simulink model "fw_can1_codec"  (R2026b)
settings: Solver=VariableStepAuto
undefined symbols (not defined in the file or in its folder): P, Ts
libraries: simulink x4
settings Model: Creator=aomar  LastModifiedBy=aomar

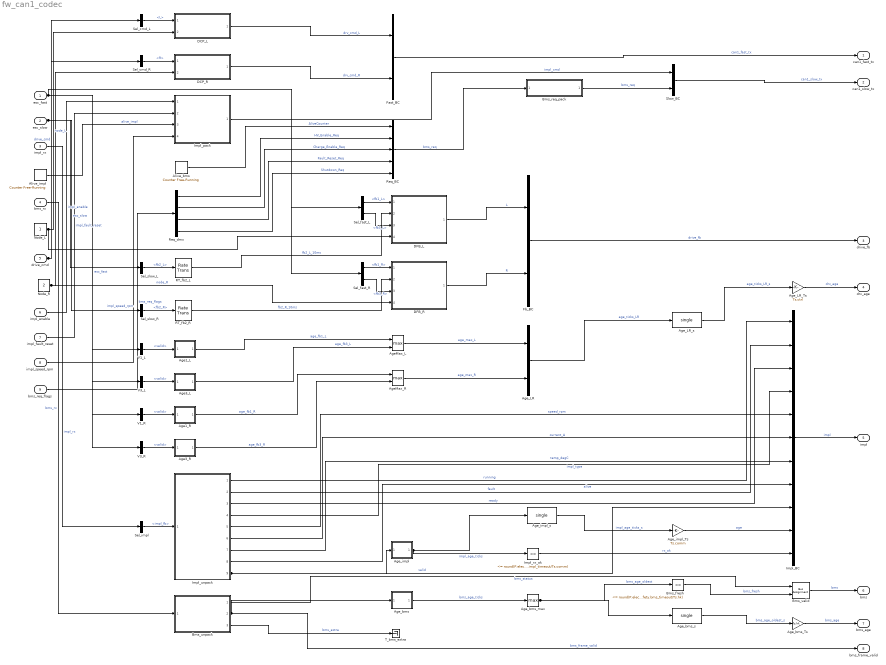
== system fw_can1_codec ==
  esc_fast : Inport  OutDataTypeStr=Bus: Bus_Can1_EscFast  SampleTime=Ts.ctrl
  esc_slow : Inport  Port=2  OutDataTypeStr=Bus: Bus_Can1_EscSlow  SampleTime=Ts.comm
  impl_rx : Inport  Port=3  OutDataTypeStr=Bus: Bus_Can1_Impl  SampleTime=Ts.comm
  bms_rx : Inport  Port=4  OutDataTypeStr=Bus: Bus_Can1_Bms  SampleTime=Ts.hk
  drive_cmd : Inport  Port=5  OutDataTypeStr=Bus: Bus_DriveCmd  SampleTime=Ts.ctrl
  impl_enable : Inport  Port=6  OutDataTypeStr=boolean  SampleTime=Ts.comm
  impl_fault_reset : Inport  Port=7  OutDataTypeStr=boolean  SampleTime=Ts.comm
  impl_speed_rpm : Inport  Port=8  OutDataTypeStr=single  SampleTime=Ts.comm
  bms_req_flags : Inport  Port=9  OutDataTypeStr=boolean  PortDimensions=4  SampleTime=Ts.comm
  Age1_L : Subsystem
  Age1_R : Subsystem
  Age3_L : Subsystem
  Age3_R : Subsystem
  AgeMax_L : MinMax  Function=max  Inputs=2
  AgeMax_R : MinMax  Function=max  Inputs=2
  Age_LR : Concatenate
  Age_LR_Ts : Gain  Gain=Ts.ctrl
  Age_LR_s : DataTypeConversion  OutDataTypeStr=single  RndMeth=Round
  Age_bms : Subsystem
  Age_bms_Ts : Gain  Gain=Ts.hk
  Age_bms_max : MinMax  Function=max
  Age_bms_s : DataTypeConversion  OutDataTypeStr=single  RndMeth=Round
  Age_impl : Subsystem
  Age_impl_Ts : Gain  Gain=Ts.comm
  Age_impl_s : DataTypeConversion  OutDataTypeStr=single  RndMeth=Round
  Alive_bms : simulink/Sources/Counter Free-Running  NumBits=8  tsamp=Ts.comm
  Alive_impl : simulink/Sources/Counter Free-Running  NumBits=8  tsamp=Ts.comm
  Bms_fresh : simulink/Logic and Bit Operations/Compare To Constant  relop=<=  const=round(P.electronics.safety.bms_timeout/Ts.hk)  OutDataTypeStr=boolean
  Bms_req_pack : Subsystem  ReferencedSubsystem=bmsreq_can_pack
  Bms_unpack : Subsystem  ReferencedSubsystem=bms_can_unpack
  Bms_valid : BusAssignment  AssignedSignals=valid
  DCP_L : Subsystem  ReferencedSubsystem=drive_cmd_pack
  DCP_R : Subsystem  ReferencedSubsystem=drive_cmd_pack
  DFB_L : Subsystem  ReferencedSubsystem=drive_fb_unpack
  DFB_R : Subsystem  ReferencedSubsystem=drive_fb_unpack
  Fast_BC : BusCreator  Inputs=2  OutDataTypeStr=Bus: Bus_Can1_McuFast  NonVirtualBus=on
      settings: InheritFromInputs=off
  Fb_BC : BusCreator  Inputs=2  OutDataTypeStr=Bus: Bus_DriveFb  NonVirtualBus=on
      settings: InheritFromInputs=off
  Impl_BC : BusCreator  Inputs=11
  Impl_pack : Subsystem  ReferencedSubsystem=implcmd_can_pack
  Impl_rx_ok : simulink/Logic and Bit Operations/Compare To Constant  relop=<=  const=round(P.electronics.safety.impl_timeout/Ts.comm)  OutDataTypeStr=boolean
  Impl_unpack : Subsystem  ReferencedSubsystem=implfb_can_unpack
  Node_L : Constant  OutDataTypeStr=uint8  SampleTime=-1
  Node_R : Constant  Value=2  OutDataTypeStr=uint8  SampleTime=-1
  RT_fb2_L : RateTransition  InitialCondition=P.ic.Bus_CanFrame8  OutPortSampleTime=Ts.ctrl
  RT_fb2_R : RateTransition  InitialCondition=P.ic.Bus_CanFrame8  OutPortSampleTime=Ts.ctrl
  Req_BC : BusCreator  Inputs=5  OutDataTypeStr=Bus: Bus_BmsReq  NonVirtualBus=on
      settings: InheritFromInputs=off
  Req_dmx : Demux
  Sel_cmd_L : BusSelector  OutputSignals=L
  Sel_cmd_R : BusSelector  OutputSignals=R
  Sel_fast_L : BusSelector  OutputSignals=fb1_L,fb3_L
  Sel_fast_R : BusSelector  OutputSignals=fb1_R,fb3_R
  Sel_impl : BusSelector  OutputSignals=impl_fb
  Sel_slow_L : BusSelector  OutputSignals=fb2_L
  Sel_slow_R : BusSelector  OutputSignals=fb2_R
  Slow_BC : BusCreator  Inputs=2  OutDataTypeStr=Bus: Bus_Can1_McuSlow  NonVirtualBus=on
      settings: InheritFromInputs=off
  T_bms_extra : Terminator
  V1_L : BusSelector  OutputSignals=fb1_L.valid
  V1_R : BusSelector  OutputSignals=fb1_R.valid
  V3_L : BusSelector  OutputSignals=fb3_L.valid
  V3_R : BusSelector  OutputSignals=fb3_R.valid
  can1_fast_tx : Outport  OutDataTypeStr=Bus: Bus_Can1_McuFast
  can1_slow_tx : Outport  Port=2  OutDataTypeStr=Bus: Bus_Can1_McuSlow
  drive_fb : Outport  Port=3  OutDataTypeStr=Bus: Bus_DriveFb
  drv_age : Outport  Port=4  OutDataTypeStr=single
  impl : Outport  Port=5
  bms : Outport  Port=6  OutDataTypeStr=Bus: Bus_BmsStatus
  bms_age : Outport  Port=7  OutDataTypeStr=single
  bms_frame_valid : Outport  Port=8  OutDataTypeStr=boolean
  wires:
  esc_fast/1 -> V3_R/1, V1_R/1, V3_L/1, V1_L/1, Sel_fast_R/1, Sel_fast_L/1  "esc_fast"
  esc_slow/1 -> Sel_slow_R/1, Sel_slow_L/1  "esc_slow"
  impl_rx/1 -> Sel_impl/1  "impl_rx"
  Alive_impl/1 -> Impl_pack/3  "alive_impl"
  bms_rx/1 -> Bms_unpack/1  "bms_rx"
  Node_L/1 -> DCP_L/2, DFB_L/4  "node_L"
  drive_cmd/1 -> Sel_cmd_L/1, Sel_cmd_R/1  "drive_cmd"
  impl_enable/1 -> Impl_pack/1  "impl_enable"
  impl_fault_reset/1 -> Impl_pack/2  "impl_fault_reset"
  impl_speed_rpm/1 -> Impl_pack/4  "impl_speed_rpm"
  bms_req_flags/1 -> Req_dmx/1  "bms_req_flags"
  Node_R/1 -> DCP_R/2, DFB_R/4  "node_R"
  Sel_cmd_L/1 -> DCP_L/1  "<L>"
  Sel_cmd_R/1 -> DCP_R/1  "<R>"
  Sel_slow_L/1 -> RT_fb2_L/1  "<fb2_L>"
  Sel_slow_R/1 -> RT_fb2_R/1  "<fb2_R>"
  V1_L/1 -> Age1_L/1(fresh)  "<valid>"
  V3_L/1 -> Age3_L/1(fresh)  "<valid>"
  V1_R/1 -> Age1_R/1(fresh)  "<valid>"
  V3_R/1 -> Age3_R/1(fresh)  "<valid>"
  Sel_impl/1 -> Impl_unpack/1  "<impl_fb>"
  Req_dmx/1 -> Req_BC/2  "HV_Enable_Req"
  Req_dmx/2 -> Req_BC/3  "Charge_Enable_Req"
  Req_dmx/3 -> Req_BC/4  "Fault_Reset_Req"
  Req_dmx/4 -> Req_BC/5  "Shutdown_Req"
  Alive_bms/1 -> Req_BC/1  "AliveCounter"
  RT_fb2_L/1 -> DFB_L/2  "fb2_L_10ms"
  RT_fb2_R/1 -> DFB_R/2  "fb2_R_10ms"
  Age1_L/1(ticks) -> AgeMax_L/1  "age_fb1_L"
  Age3_L/1(ticks) -> AgeMax_L/2  "age_fb3_L"
  Age1_R/1(ticks) -> AgeMax_R/1  "age_fb1_R"
  Age3_R/1(ticks) -> AgeMax_R/2  "age_fb3_R"
  DCP_L/1 -> Fast_BC/1  "drv_cmd_L"
  DCP_R/1 -> Fast_BC/2  "drv_cmd_R"
  Impl_pack/1 -> Slow_BC/1  "impl_cmd"
  Impl_unpack/1 -> Impl_BC/1  "running"
  Impl_unpack/2 -> Impl_BC/2  "fault"
  Impl_unpack/3 -> Impl_BC/3  "ready"
  Impl_unpack/4 -> Impl_BC/4  "impl_type"
  Impl_unpack/5 -> Impl_BC/5  "speed_rpm"
  Impl_unpack/6 -> Impl_BC/6  "current_A"
  Impl_unpack/7 -> Impl_BC/7  "temp_degC"
  Impl_unpack/8 -> Impl_BC/8  "alive"
  Impl_unpack/9 -> Impl_BC/9, Age_impl/1(fresh)  "valid"
  Bms_unpack/1 -> Bms_valid/1  "bms_status"
  Bms_unpack/2 -> bms_frame_valid/1, Age_bms/1(fresh)  "bms_frame_valid"
  Bms_unpack/3 -> T_bms_extra/1  "bms_extra"
  Sel_fast_L/1 -> DFB_L/1  "<fb1_L>"
  Sel_fast_L/2 -> DFB_L/3  "<fb3_L>"
  Sel_fast_R/1 -> DFB_R/1  "<fb1_R>"
  Sel_fast_R/2 -> DFB_R/3  "<fb3_R>"
  Fast_BC/1 -> can1_fast_tx/1  "can1_fast_tx"
  Req_BC/1 -> Bms_req_pack/1  "bms_req"
  AgeMax_L/1 -> Age_LR/1  "age_max_L"
  AgeMax_R/1 -> Age_LR/2  "age_max_R"
  Age_impl/1(ticks) -> Age_impl_s/1, Impl_rx_ok/1  "impl_age_ticks"
  Age_bms/1(ticks) -> Age_bms_max/1  "bms_age_ticks"
  DFB_L/1 -> Fb_BC/1  "L"
  DFB_R/1 -> Fb_BC/2  "R"
  Fb_BC/1 -> drive_fb/1  "drive_fb"
  Age_LR/1 -> Age_LR_s/1  "age_ticks_LR"
  Impl_rx_ok/1 -> Impl_BC/11  "rx_ok"
  Age_bms_max/1 -> Bms_fresh/1, Age_bms_s/1  "bms_age_oldest"
  Age_impl_s/1 -> Age_impl_Ts/1  "impl_age_ticks_s"
  Bms_req_pack/1 -> Slow_BC/2  "bms_req"
  Slow_BC/1 -> can1_slow_tx/1  "can1_slow_tx"
  Age_impl_Ts/1 -> Impl_BC/10  "age"
  Bms_fresh/1 -> Bms_valid/2  "bms_fresh"
  Age_LR_s/1 -> Age_LR_Ts/1  "age_ticks_LR_s"
  Age_bms_s/1 -> Age_bms_Ts/1  "bms_age_oldest_s"
  Impl_BC/1 -> impl/1  "impl"
  Age_LR_Ts/1 -> drv_age/1  "drv_age"
  Age_bms_Ts/1 -> bms_age/1  "bms_age"
  Bms_valid/1 -> bms/1  "bms"

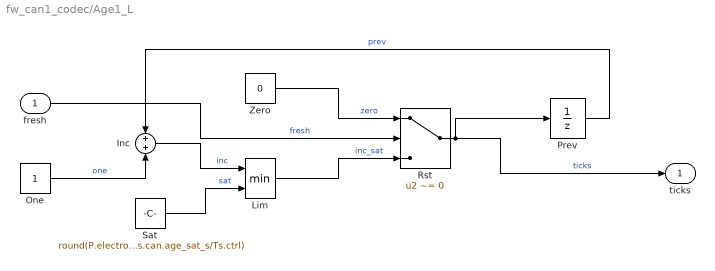
== system fw_can1_codec/Age1_L ==
  fresh : Inport
  Inc : Sum  OutDataTypeStr=uint16  SaturateOnIntegerOverflow=on
  Lim : MinMax  Inputs=2
  One : Constant  OutDataTypeStr=uint16  SampleTime=-1
  Prev : UnitDelay  InitialCondition=round(P.electronics.can.age_sat_s/Ts.ctrl)  SampleTime=-1
  Rst : Switch  Criteria=u2 ~= 0  SaturateOnIntegerOverflow=off  InputSameDT=off
  Sat : Constant  Value=round(P.electronics.can.age_sat_s/Ts.ctrl)  OutDataTypeStr=uint16  SampleTime=-1
  Zero : Constant  Value=0  OutDataTypeStr=uint16  SampleTime=-1
  ticks : Outport
  wires:
  fresh/1 -> Rst/2  "fresh"
  One/1 -> Inc/2  "one"
  Inc/1 -> Lim/1  "inc"
  Sat/1 -> Lim/2  "sat"
  Zero/1 -> Rst/1  "zero"
  Lim/1 -> Rst/3  "inc_sat"
  Rst/1 -> ticks/1, Prev/1  "ticks"
  Prev/1 -> Inc/1  "prev"

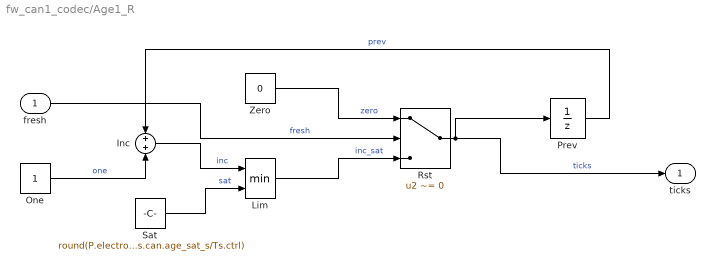
== system fw_can1_codec/Age1_R ==
  fresh : Inport
  Inc : Sum  OutDataTypeStr=uint16  SaturateOnIntegerOverflow=on
  Lim : MinMax  Inputs=2
  One : Constant  OutDataTypeStr=uint16  SampleTime=-1
  Prev : UnitDelay  InitialCondition=round(P.electronics.can.age_sat_s/Ts.ctrl)  SampleTime=-1
  Rst : Switch  Criteria=u2 ~= 0  SaturateOnIntegerOverflow=off  InputSameDT=off
  Sat : Constant  Value=round(P.electronics.can.age_sat_s/Ts.ctrl)  OutDataTypeStr=uint16  SampleTime=-1
  Zero : Constant  Value=0  OutDataTypeStr=uint16  SampleTime=-1
  ticks : Outport
  wires:
  fresh/1 -> Rst/2  "fresh"
  One/1 -> Inc/2  "one"
  Inc/1 -> Lim/1  "inc"
  Sat/1 -> Lim/2  "sat"
  Zero/1 -> Rst/1  "zero"
  Lim/1 -> Rst/3  "inc_sat"
  Rst/1 -> ticks/1, Prev/1  "ticks"
  Prev/1 -> Inc/1  "prev"

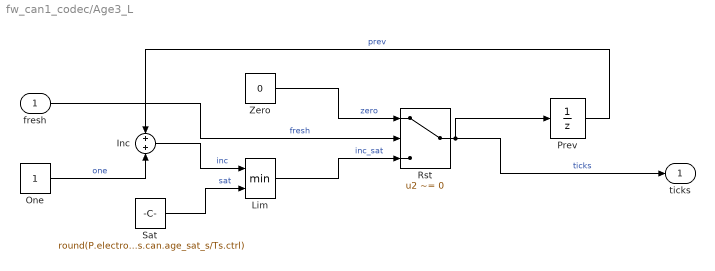
== system fw_can1_codec/Age3_L ==
  fresh : Inport
  Inc : Sum  OutDataTypeStr=uint16  SaturateOnIntegerOverflow=on
  Lim : MinMax  Inputs=2
  One : Constant  OutDataTypeStr=uint16  SampleTime=-1
  Prev : UnitDelay  InitialCondition=round(P.electronics.can.age_sat_s/Ts.ctrl)  SampleTime=-1
  Rst : Switch  Criteria=u2 ~= 0  SaturateOnIntegerOverflow=off  InputSameDT=off
  Sat : Constant  Value=round(P.electronics.can.age_sat_s/Ts.ctrl)  OutDataTypeStr=uint16  SampleTime=-1
  Zero : Constant  Value=0  OutDataTypeStr=uint16  SampleTime=-1
  ticks : Outport
  wires:
  fresh/1 -> Rst/2  "fresh"
  One/1 -> Inc/2  "one"
  Inc/1 -> Lim/1  "inc"
  Sat/1 -> Lim/2  "sat"
  Zero/1 -> Rst/1  "zero"
  Lim/1 -> Rst/3  "inc_sat"
  Rst/1 -> ticks/1, Prev/1  "ticks"
  Prev/1 -> Inc/1  "prev"

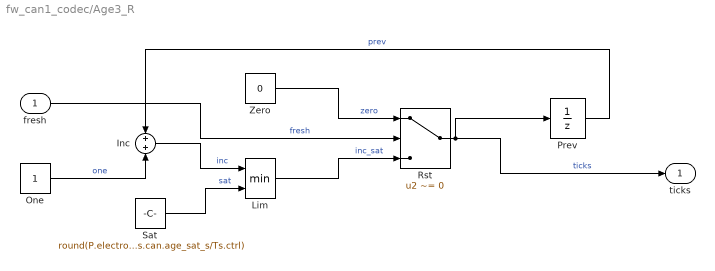
== system fw_can1_codec/Age3_R ==
  fresh : Inport
  Inc : Sum  OutDataTypeStr=uint16  SaturateOnIntegerOverflow=on
  Lim : MinMax  Inputs=2
  One : Constant  OutDataTypeStr=uint16  SampleTime=-1
  Prev : UnitDelay  InitialCondition=round(P.electronics.can.age_sat_s/Ts.ctrl)  SampleTime=-1
  Rst : Switch  Criteria=u2 ~= 0  SaturateOnIntegerOverflow=off  InputSameDT=off
  Sat : Constant  Value=round(P.electronics.can.age_sat_s/Ts.ctrl)  OutDataTypeStr=uint16  SampleTime=-1
  Zero : Constant  Value=0  OutDataTypeStr=uint16  SampleTime=-1
  ticks : Outport
  wires:
  fresh/1 -> Rst/2  "fresh"
  One/1 -> Inc/2  "one"
  Inc/1 -> Lim/1  "inc"
  Sat/1 -> Lim/2  "sat"
  Zero/1 -> Rst/1  "zero"
  Lim/1 -> Rst/3  "inc_sat"
  Rst/1 -> ticks/1, Prev/1  "ticks"
  Prev/1 -> Inc/1  "prev"

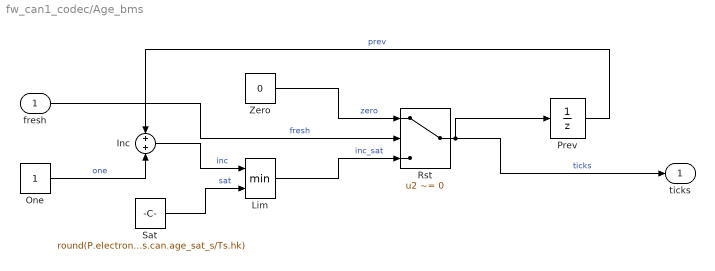
== system fw_can1_codec/Age_bms ==
  fresh : Inport
  Inc : Sum  OutDataTypeStr=uint16  SaturateOnIntegerOverflow=on
  Lim : MinMax  Inputs=2
  One : Constant  OutDataTypeStr=uint16  SampleTime=-1
  Prev : UnitDelay  InitialCondition=round(P.electronics.can.age_sat_s/Ts.hk)  SampleTime=-1
  Rst : Switch  Criteria=u2 ~= 0  SaturateOnIntegerOverflow=off  InputSameDT=off
  Sat : Constant  Value=round(P.electronics.can.age_sat_s/Ts.hk)  OutDataTypeStr=uint16  SampleTime=-1
  Zero : Constant  Value=0  OutDataTypeStr=uint16  SampleTime=-1
  ticks : Outport
  wires:
  fresh/1 -> Rst/2  "fresh"
  One/1 -> Inc/2  "one"
  Inc/1 -> Lim/1  "inc"
  Sat/1 -> Lim/2  "sat"
  Zero/1 -> Rst/1  "zero"
  Lim/1 -> Rst/3  "inc_sat"
  Rst/1 -> ticks/1, Prev/1  "ticks"
  Prev/1 -> Inc/1  "prev"

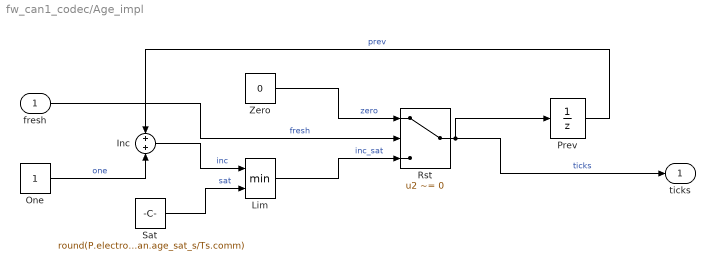
== system fw_can1_codec/Age_impl ==
  fresh : Inport
  Inc : Sum  OutDataTypeStr=uint16  SaturateOnIntegerOverflow=on
  Lim : MinMax  Inputs=2
  One : Constant  OutDataTypeStr=uint16  SampleTime=-1
  Prev : UnitDelay  InitialCondition=round(P.electronics.can.age_sat_s/Ts.comm)  SampleTime=-1
  Rst : Switch  Criteria=u2 ~= 0  SaturateOnIntegerOverflow=off  InputSameDT=off
  Sat : Constant  Value=round(P.electronics.can.age_sat_s/Ts.comm)  OutDataTypeStr=uint16  SampleTime=-1
  Zero : Constant  Value=0  OutDataTypeStr=uint16  SampleTime=-1
  ticks : Outport
  wires:
  fresh/1 -> Rst/2  "fresh"
  One/1 -> Inc/2  "one"
  Inc/1 -> Lim/1  "inc"
  Sat/1 -> Lim/2  "sat"
  Zero/1 -> Rst/1  "zero"
  Lim/1 -> Rst/3  "inc_sat"
  Rst/1 -> ticks/1, Prev/1  "ticks"
  Prev/1 -> Inc/1  "prev"
